simulink model "furuta_single_inverted_deploy"  (R2025a)
settings: Solver=FixedStepDiscrete  StartTime=0.0  StopTime=inf  FixedStep=Ts  RelTol=1e-3
InitFcn:
  | addpath('functions');
model workspace (MATLAB code in the model file):
  | arm_torque = 0;
  | L_arm = 0.2;
  | I_arm = 0.01;
  | lcom_1 = 0.6;
  | I_1 = 0.02;
  | m_1 = 1;
  | L_1 = 1;
  | 
  | init_cond = [pi/2; 0; 0.01; 0];
undefined symbols (not defined in the file or in its folder): DiscIntNeverNeededParam, Kd_PendulumAngle, Ts
libraries: simulink x1
settings Model: Creator=Esther  LastModifiedBy=31215

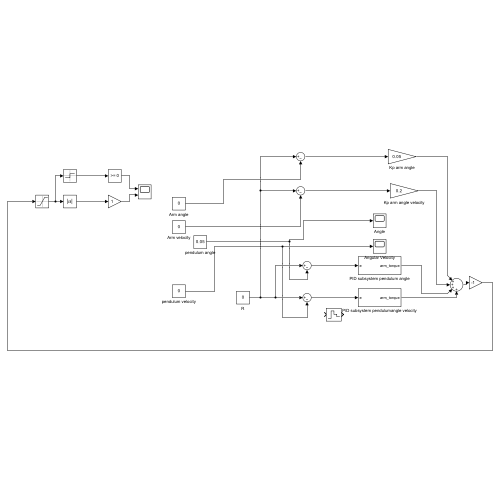
[thumbnail: Simulink's stored preview of the top-level diagram]
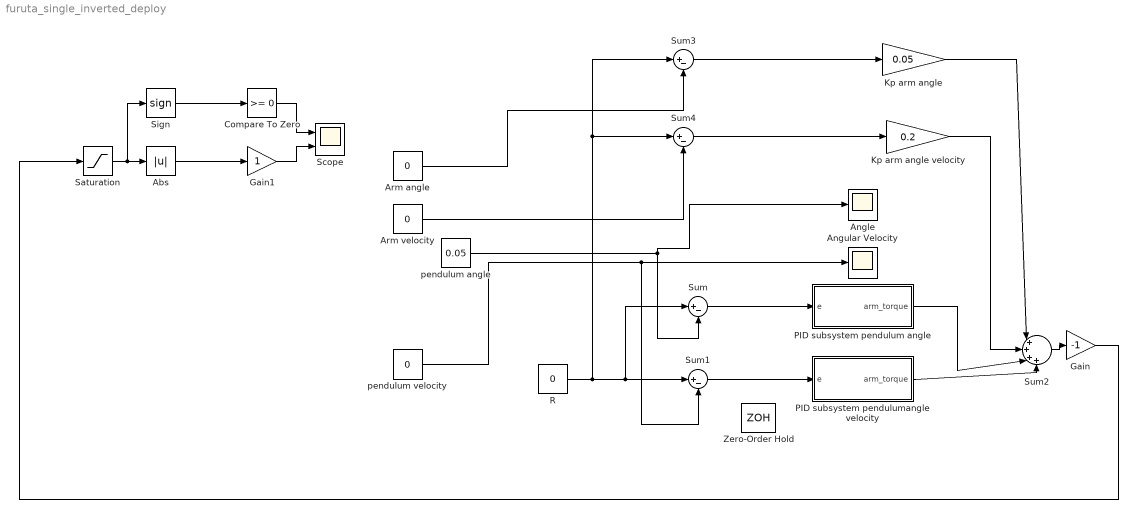
== system furuta_single_inverted_deploy ==
  Abs : Abs  SaturateOnIntegerOverflow=off
  Angle : Scope
      settings: ActiveDisplayYMinimum=-6.9679733150236753  ActiveDisplayYMaximum=4.0512303756780108
  Angular Velocity : Scope
      settings: ActiveDisplayYMinimum=-3875.8658390527003  ActiveDisplayYMaximum=3642.7464695660938  DataLoggingVariableName=ScopeData2
  Arm angle : Constant  Value=0
  Arm velocity : Constant  Value=0
  Compare To Zero : simulink/Logic and Bit Operations/Compare To Zero  relop=>=  OutDataTypeStr=boolean
  Gain : Gain  Gain=-1
  Gain1 : Gain
  Kp arm angle : Gain  Gain=0.05
  Kp arm angle velocity : Gain  Gain=0.2
  PID subsystem pendulum angle : Subsystem
  PID subsystem pendulumangle velocity : Subsystem
  R : Constant  Value=0
  Saturation : Saturate
  Scope : Scope  NumInputPorts=2
      settings: ActiveDisplayYMinimum=0.4375  ActiveDisplayYMaximum=1.0625
  Sign : Signum
  Sum{,1,3..4} (4 alike) : Sum  Inputs=|+-
  Sum2 : Sum  Inputs=|++++
  Zero-Order Hold : ZeroOrderHold  SampleTime=Ts
  pendulum angle : Constant  Value=0.05
  pendulum velocity : Constant  Value=0
  wires:
  R/1 -> Sum4/1, Sum3/1, Sum1/1, Sum/1
  pendulum angle/1 -> Sum/2, Angle/1
  pendulum velocity/1 -> Angular Velocity/1, Sum1/2
  Sum/1 -> PID subsystem pendulum angle/1(e)
  Sum2/1 -> Gain/1
  Gain/1 -> Saturation/1
  Kp arm angle velocity/1 -> Sum2/2
  Kp arm angle/1 -> Sum2/1
  PID subsystem pendulum angle/1(arm_torque) -> Sum2/3
  Arm angle/1 -> Sum3/2
  Arm velocity/1 -> Sum4/2
  Sum3/1 -> Kp arm angle/1
  Sum4/1 -> Kp arm angle velocity/1
  Saturation/1 -> Sign/1, Abs/1
  Abs/1 -> Gain1/1
  Sign/1 -> Compare To Zero/1
  Compare To Zero/1 -> Scope/1
  Gain1/1 -> Scope/2
  Sum1/1 -> PID subsystem pendulumangle velocity/1(e)
  PID subsystem pendulumangle velocity/1(arm_torque) -> Sum2/4

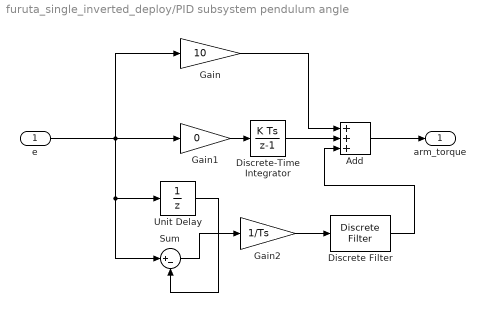
== system furuta_single_inverted_deploy/PID subsystem pendulum angle ==
  e : Inport
  Add : Sum  Inputs=+++
  Discrete Filter : DiscreteFilter
  Discrete-Time Integrator : DiscreteIntegrator  gainval=1  SampleTime=0.001  ICPrevOutput=DiscIntNeverNeededParam  ICPrevScaledInput=DiscIntNeverNeededParam
  Gain : Gain  Gain=10
  Gain1 : Gain  Gain=0
  Gain2 : Gain  Gain=1/Ts
  Sum : Sum  Inputs=|+-
  Unit Delay : UnitDelay  SampleTime=-1  HasFrameUpgradeWarning=on
  arm_torque : Outport
  wires:
  e/1 -> Sum/1, Unit Delay/1, Gain/1, Gain1/1
  Gain1/1 -> Discrete-Time Integrator/1
  Gain/1 -> Add/1
  Discrete-Time Integrator/1 -> Add/2
  Add/1 -> arm_torque/1
  Unit Delay/1 -> Sum/2
  Sum/1 -> Gain2/1
  Gain2/1 -> Discrete Filter/1
  Discrete Filter/1 -> Add/3

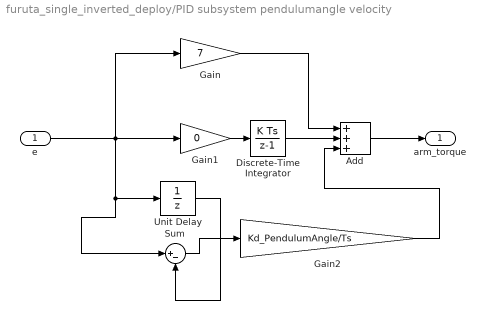
== system furuta_single_inverted_deploy/PID subsystem pendulumangle velocity ==
  e : Inport
  Add : Sum  Inputs=+++
  Discrete-Time Integrator : DiscreteIntegrator  gainval=1  SampleTime=0.001  ICPrevOutput=DiscIntNeverNeededParam  ICPrevScaledInput=DiscIntNeverNeededParam
  Gain : Gain  Gain=7
  Gain1 : Gain  Gain=0
  Gain2 : Gain  Gain=Kd_PendulumAngle/Ts
  Sum : Sum  Inputs=|+-
  Unit Delay : UnitDelay  SampleTime=-1  HasFrameUpgradeWarning=on
  arm_torque : Outport
  wires:
  Sum/1 -> Gain2/1
  Unit Delay/1 -> Sum/2
  Gain1/1 -> Discrete-Time Integrator/1
  Gain2/1 -> Add/3
  Discrete-Time Integrator/1 -> Add/2
  Add/1 -> arm_torque/1
  Gain/1 -> Add/1
  e/1 -> Sum/1, Unit Delay/1, Gain/1, Gain1/1
